simulink model "TestModel_V5_Timing_V2_2024a"  (R2024a)
settings: Solver=FixedStepAuto  StartTime=0.0  StopTime=40  FixedStep=1e-6  RelTol=1e-3
values from neighbouring files (symbols this model uses):
  par_Ctrl_FluxOffset = 0    [Param.m]
  par_Ctrl_MI = 0.99    [Param.m]
  par_Ctrl_SpdRt = 10    [Param.m]
  par_Ctrl_ThetaOffset = 0    [Param.m]
  par_IM_Frated = 50    [Param.m]
  par_IM_IratedPh = 7.9/sqrt(3)    [Param.m]
  par_IM_Lm = 0.527    [Param.m]
  par_IM_Lr = par_IM_Lm + par_IM_Llr    (= 0.5639)    [Param.m]
  par_IM_pp = 2    [Param.m]
  par_IM_Rs = 3.14    [Param.m]
  par_IM_VrmsLL = 400    [Param.m]
  par_uc_Ts = 100e-6    (= 0.0001)    [Param.m]
  pmsm = mcb.getPMSMParameters('Teknic2310P')    [mcb_pmsm_foc_sensorless_f28379d_datascript.m]
  Ts = T_pwm    (= 5e-05)    [mcb_pmsm_foc_sensorless_f28379d_datascript.m]
  Ts_motor = T_pwm/2    (= 2.5e-05)    [mcb_pmsm_foc_sensorless_f28379d_datascript.m]
undefined symbols (not defined in the file or in its folder): DiscIntNeverNeededParam, IM, par_pmsm_FluxLinkage, par_pmsm_Frated, par_pmsm_pp, par_pmsm_Vboost, par_pmsm_VrmsLL
libraries: spsOnDelayLib x24, mcbcontrolslib x12, spsTriangleGeneratorLib x4, autolibim x3, spsFirstOrderFilterLib x3, spsCurrentMeasurementLib x2, spsDCVoltageSourceLib x2, spsVoltageMeasurementLib x2, spsTwoLevelConverterLib x2, spsThreePhaseVIMeasurementLib x2, spsSeriesRLCBranchLib x1, sdolib x1
(part 1 of 3)
settings Model: PacingRate=1000  Creator=ckb527612  LastModifiedBy=ckb527612
settings ConfigComp: CovBoundaryAbsTol=1.0e-5

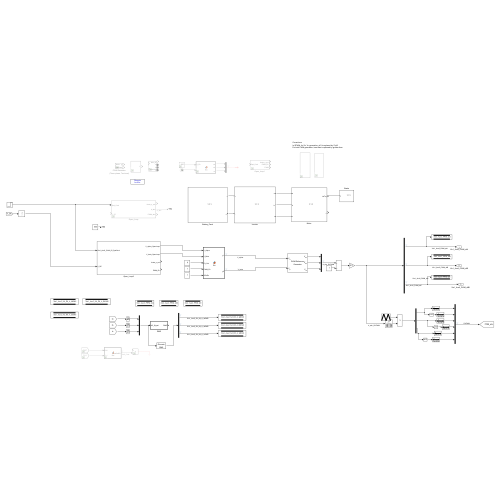
[thumbnail: Simulink's stored preview of the top-level diagram]
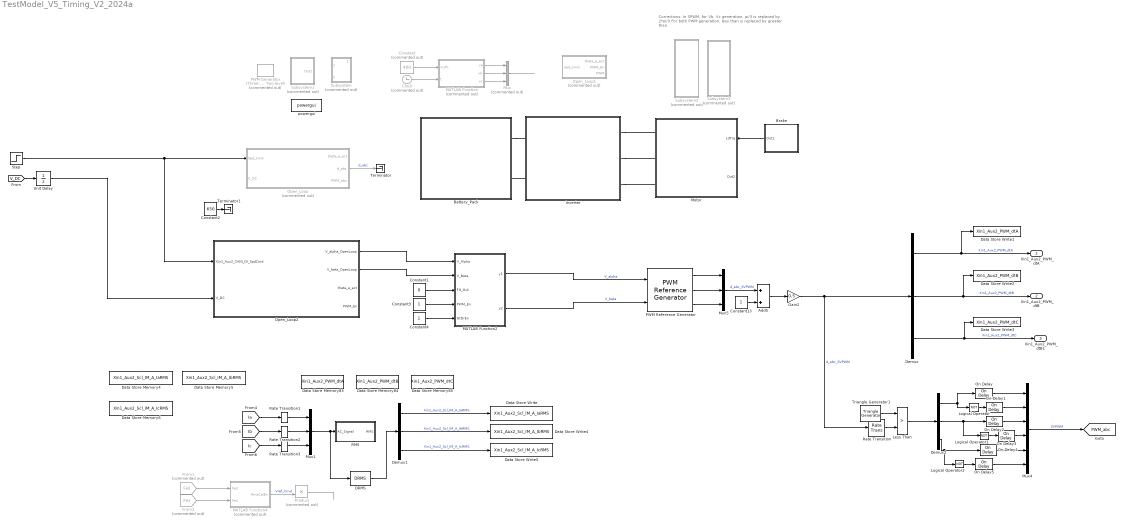
== system TestModel_V5_Timing_V2_2024a ==
  note: Corrections:
      | In SPWM, for Vb, Vc generation, pi/3 is replaced by 2*pi/3
      | For both PWM generation, less than is replaced by greater than
  Add5 : Sum
  Battery_Pack : Subsystem
      mask Display: image('battery_pack.jpg');
  Brake : Subsystem
      mask Display: image('brake-system-types-and-hydraulic-brake-parts-and-functions-6.png');
  Clock : Clock  Commented=on
  Constant : Constant  Commented=on  Value=400
  Constant1 : Constant  Value=0
  Constant13 : Constant
  Constant2 : Constant  Value=650
  Constant3 : Constant
  Constant4 : Constant
  DRMS : sdolib/RMS Blocks/DRMS  Ts=par_uc_Ts
  Data Store Memory4 : DataStoreMemory  DataStoreName=Xin1_Aux2_Scl_IM_A_IaRMS  WriteAfterWriteMsg=warning  ShowAdditionalParam=off
  Data Store Memory5 : DataStoreMemory  DataStoreName=Xin1_Aux2_Scl_IM_A_IbRMS  WriteAfterWriteMsg=warning  ShowAdditionalParam=off
  Data Store Memory6 : DataStoreMemory  DataStoreName=Xin1_Aux2_Scl_IM_A_IcRMS  WriteAfterWriteMsg=warning  ShowAdditionalParam=off
  Data Store Memory83 : DataStoreMemory  DataStoreName=Xin1_Aux2_PWM_dtA  WriteAfterWriteMsg=warning  ShowAdditionalParam=off
  Data Store Memory84 : DataStoreMemory  DataStoreName=Xin1_Aux2_PWM_dtB  WriteAfterWriteMsg=warning  ShowAdditionalParam=off
  Data Store Memory85 : DataStoreMemory  DataStoreName=Xin1_Aux2_PWM_dtC  WriteAfterWriteMsg=warning  ShowAdditionalParam=off
  Data Store Write : DataStoreWrite  DataStoreName=Xin1_Aux2_Scl_IM_A_IaRMS  IndexOptions=Index vector (dialog)  Indices=1  OutputSizes=1
  Data Store Write1 : DataStoreWrite  DataStoreName=Xin1_Aux2_PWM_dtA  IndexOptions=Index vector (dialog)  Indices=1  OutputSizes=1
  Data Store Write2 : DataStoreWrite  DataStoreName=Xin1_Aux2_PWM_dtB  IndexOptions=Index vector (dialog)  Indices=1  OutputSizes=1
  Data Store Write3 : DataStoreWrite  DataStoreName=Xin1_Aux2_PWM_dtC  IndexOptions=Index vector (dialog)  Indices=1  OutputSizes=1
  Data Store Write4 : DataStoreWrite  DataStoreName=Xin1_Aux2_Scl_IM_A_IbRMS  IndexOptions=Index vector (dialog)  Indices=1  OutputSizes=1
  Data Store Write5 : DataStoreWrite  DataStoreName=Xin1_Aux2_Scl_IM_A_IcRMS  IndexOptions=Index vector (dialog)  Indices=1  OutputSizes=1
  Demux : Demux  Outputs=3
  Demux1 : Demux  Outputs=3
  Demux2 : Demux  Outputs=3
  From1 : From  Commented=on  GotoTag=Fe2  TagVisibility=global
  From2 : From  Commented=on  GotoTag=Fe1  TagVisibility=global
  Gain2 : Gain  Gain=0.5
  Inverter : Subsystem
      mask Display: image('inverter.jpg');
  Less Than : RelationalOperator  Operator=>  OutDataTypeStr=boolean  RndMeth=Simplest  InputSameDT=off
  Logical Operator : Logic  Operator=NOT  AllPortsSameDT=off  OutDataTypeStr=boolean
  Logical Operator1 : Logic  Operator=NOT  AllPortsSameDT=off  OutDataTypeStr=boolean
  Logical Operator2 : Logic  Operator=NOT  AllPortsSameDT=off  OutDataTypeStr=boolean
  MATLAB Function : MATLAB Function  Commented=on  TreatAsAtomicUnit=on
  MATLAB Function2 : MATLAB Function  TreatAsAtomicUnit=on
  MATLAB Function4 : MATLAB Function  Commented=on  TreatAsAtomicUnit=on
  Motor : Subsystem
      settings: PortSchema="{\"entries\":[{\"content\":{\"sides\":[{\"content\":{\"connectorIds\":[\"LConn1\",\"LConn2\",\"LConn3\"]},\"type\":\"ConnectorPlacement.EquallySpacedRectSide\",\"uuid\":\"ba224176-031b-46fb-9c66-bda2665a14bd\"},{\"content\":{\"connectorIds\":[\"In1\",\"Out1\"],\"side\":\"RIGHT\"},\"type\":\"ConnectorPlacement.EquallySpacedRectSide\",\"uuid\":\"afd0beac-69db-400a-8bb3-39f53f6dd0dc\"},{\"content\":{\"side\":\"TOP\"},\"type\":\"ConnectorPlacement.EquallySpacedRectSide\",\"uuid\":\"9d949d83-5907-4238-9cb9-0d10379fcdec\"}]},\"type\":\"ConnectorPlacement.EquallySpacedConnector\",\"uuid\":\"43d01ac6-0c0f-4af8-b336-a00f131902fe\"}],\"packageUris\":[\"http://schema.mathworks.com/mf0/Connector/R2020b\"],\"version\":\"1.0\"}"
      mask Display: image('Motor3.jpg');
  Mux : Mux  Commented=on  Inputs=3
  Mux1 : Mux  Inputs=3
  Mux4 : Mux  Inputs=6
  Mux5 : Mux  Inputs=3
  On Delay{,1..5} (6 alike) : spsOnDelayLib/On Delay  DelayType=On delay  delay=3e-6  ic=0  Ts=1e-6
  Open_Loop : Subsystem  Commented=on
  Open_Loop1 : Subsystem  Commented=on
  Open_Loop2 : Subsystem
  "PWM Generator (Three-phase, Two-level)" : eePwmGeneratorTwoLevel/PWM Generator (Three-phase, Two-level)  Commented=on  PWMMode=Continuous PWM (CPWM)  CPWMMode=SVM: space vector modulation  DPWMMode=60 DPWM: 60 degree discontinuous PWM  fsw=10e3  Ts=1e-6
      settings: LibrarySourceBlock=|
      | ee_sl_lib/Pulse Width
      | Modulation/PWM Generator
      | (Three-phase, Two-level)
  PWM Reference Generator : mcbcontrolslib/PWM Reference Generator  inSignal=Valphabeta  modType=SVM: space vector modulation
      settings: LibrarySourceBlock=mcbhdllib/Controls/Math Transforms/PWM Reference Generator
  Product : Product  Commented=on
  RMS : Subsystem  TreatAsAtomicUnit=on
  Rate Transition : RateTransition
  Rate Transition1 : RateTransition  OutPortSampleTime=par_uc_Ts
  Rate Transition2 : RateTransition  OutPortSampleTime=par_uc_Ts
  Rate Transition3 : RateTransition  OutPortSampleTime=par_uc_Ts
  Step : Step  After=500
  Subsystem : Subsystem  Commented=on
  Subsystem1 : Subsystem  Commented=on
  Subsystem2 : Subsystem  Commented=on
  Subsystem3 : Subsystem  Commented=on
  Terminator : Terminator
  Terminator1 : Terminator
  Triangle Generator1 : spsTriangleGeneratorLib/Triangle Generator  Freq=10e3  Phase=0  Ts=1e-6
  Unit Delay : UnitDelay  SampleTime=-1  HasFrameUpgradeWarning=on
  powergui : spspowerguiLib/powergui  Priority=1  SimulationMode=Discrete  SampleTime=1e-6  frequency=60  Iterations=50  frequencyindice=0  Pbase=100e6  ErrMax=1e-4  UnitsV=kV  UnitsW=MW  buscounter=0  FunctionMessages=off  echomessages=off  EnableUseOfTLC=off  CurrentSourceSwitches=off  DisableSnubberDevices=off  DisableRonSwitches=off  DisableVfSwitches=off  DisplayEquations=off  AutomaticDiscreteSolvers=off  SolverType=Tustin/Backward Euler (TBE)  Interpol=off  ExternalGateDelay=off  methode=off  Ts=100  x0status=blocks  SPID=on  SwTol=0  HookPort=off  NonlinearTolerance=1e-4  nMaxIteration=100  ContinueOnMaxIteration=off  RestoreLinks=warning  ResistiveCurrentMeasurement=off  Frange=[0:2:500]  Ylog=off  Xlog=on  ShowGrid=off  save=off  variable=ZData  structure=0  ZoomFFT=off  StartTime=0.0  cycles=1  DisplayStyle=1  fundamental=60  FreqAxis=off  MaxFrequency=1000  frequencyindicesteady=1  RmsSteady=1  display=off
  Xin1_Aux2_PWM_dtA : Outport  VectorParamsAs1DForOutWhenUnconnected=off
  Xin1_Aux2_PWM_dtB : Outport  Port=2  VectorParamsAs1DForOutWhenUnconnected=off
  Xin1_Aux2_PWM_dtB1 : Outport  Port=3  VectorParamsAs1DForOutWhenUnconnected=off
  tag scope: PWM_abc=global
  wires:
  Constant/1 -> MATLAB Function/1(V_Ph)
  MATLAB Function/1(va) -> Mux/1
  MATLAB Function/2(vb) -> Mux/2
  MATLAB Function/3(vc) -> Mux/3
  Mux/1 -> ?
  Clock/1 -> MATLAB Function/2(t)
  Brake/1(Out1) -> Motor/1(LdTrq)
  Constant2/1 -> Terminator1/1
  Open_Loop/2(d_abc) -> Terminator/1  "d_abc"
  [V_DC] -> Unit Delay/1
  Unit Delay/1 -> Open_Loop2/2(V_DC)
  Step/1 -> Open_Loop2/1(Xin1_Aux2_CANI_DI_SpdCmd), Open_Loop/1(Spd_Cmd)
  MATLAB Function2/1(y1) -> PWM Reference Generator/1  "V_alpha"
  Constant3/1 -> MATLAB Function2/4(PWM_En)
  Constant13/1 -> Add5/2
  MATLAB Function2/2(y2) -> PWM Reference Generator/2  "V_beta"
  Demux/2 -> Data Store Write2/1, Xin1_Aux2_PWM_dtB/1  "Xin1_Aux2_PWM_dtB"
  Add5/1 -> Gain2/1
  Demux/3 -> Xin1_Aux2_PWM_dtB1/1, Data Store Write3/1  "Xin1_Aux2_PWM_dtC"
  Constant1/1 -> MATLAB Function2/3(Flt_Out)
  PWM Reference Generator/3 -> Mux5/3
  Open_Loop2/1(V_alpha_OpenLoop) -> MATLAB Function2/1(V_Alpha)
  Mux5/1 -> Add5/1  "d_abc_SVPWM"
  Open_Loop2/2(V_beta_OpenLoop) -> MATLAB Function2/2(V_Beta)
  PWM Reference Generator/2 -> Mux5/2
  Constant4/1 -> MATLAB Function2/5(GtDrEn)
  Demux/1 -> Data Store Write1/1, Xin1_Aux2_PWM_dtA/1  "Xin1_Aux2_PWM_dtA"
  PWM Reference Generator/1 -> Mux5/1
  [Ia] -> Rate Transition1/1
  [Ib] -> Rate Transition2/1
  Mux1/1 -> DRMS/1, RMS/1(AC_Signal)
  Demux1/1 -> Data Store Write/1  "Xin1_Aux2_Scl_IM_A_IaRMS"
  Demux1/3 -> Data Store Write5/1  "Xin1_Aux2_Scl_IM_A_IcRMS"
  [Ic] -> Rate Transition3/1
  DRMS/1 -> Demux1/1
  Demux1/2 -> Data Store Write4/1  "Xin1_Aux2_Scl_IM_A_IbRMS"
  Mux4/1 -> [PWM_abc]  "SVPWM"
  Logical Operator2/1 -> On Delay5/1
  On Delay5/1 -> Mux4/6
  Triangle Generator1/1 -> Less Than/1
  On Delay4/1 -> Mux4/5
  On Delay1/1 -> Mux4/2
  Logical Operator1/1 -> On Delay3/1
  Logical Operator/1 -> On Delay1/1
  Demux2/3 -> On Delay4/1, Logical Operator2/1
  Less Than/1 -> Demux2/1
  Demux2/1 -> Logical Operator/1, On Delay/1
  Demux2/2 -> On Delay2/1, Logical Operator1/1
  On Delay2/1 -> Mux4/3
  Gain2/1 -> Rate Transition/1, Demux/1  "d_abc_SVPWM"
  On Delay/1 -> Mux4/1
  On Delay3/1 -> Mux4/4
  Rate Transition/1 -> Less Than/2
  Rate Transition1/1 -> Mux1/1
  Rate Transition2/1 -> Mux1/2
  Rate Transition3/1 -> Mux1/3
  From1/1 -> MATLAB Function4/1(Fe2)
  From2/1 -> MATLAB Function4/2(Fe1)
  MATLAB Function4/1(RmsCalEn) -> Product/2  "Vref_Cmd"
  Product/1 -> ?
  connections:
  Inverter/LConn2 -- Battery_Pack/RConn2
  Inverter/RConn2 -- Motor/LConn2
  Inverter/RConn1 -- Motor/LConn1
  Battery_Pack/RConn1 -- Inverter/LConn1
  Inverter/RConn3 -- Motor/LConn3

== system TestModel_V5_Timing_V2_2024a/Battery_Pack ==
  Current Measurement : spsCurrentMeasurementLib/Current Measurement  PhasorSimulation=off  OutputType=Complex  PSBequivalent=0
  From : From  Commented=on  GotoTag=V_DC  TagVisibility=global
  Series RLC Branch : spsSeriesRLCBranchLib/Series RLC Branch  LConnTagsString=__new0  RConnTagsString=__new0  BranchType=RC  Resistance=0.4e-3  Inductance=1e-3  SetiL0=off  InitialCurrent=0  Capacitance=300e-6  Setx0=on  InitialVoltage=650  Measurements=None
  Terminator : Terminator
  "V_in " : spsDCVoltageSourceLib/DC Voltage Source  Amplitude=650  Measurements=None
  Voltage Measurement : spsVoltageMeasurementLib/Voltage Measurement  PhasorSimulation=off  OutputType=Complex  PSBequivalent=0
  - : PMIOPort  Side=Right
  -1 : PMIOPort  Port=2  Side=Right
  tag scope: I_in=global, V_DC=global
  wires:
  Current Measurement/1 -> [I_in]  "I_in"
  Voltage Measurement/1 -> [V_DC]  "V_DC"
  From/1 -> Terminator/1
  connections:
  Current Measurement/RConn1 -- -/RConn1
  Voltage Measurement/LConn1 -- Current Measurement/LConn1 -- "V_in "/RConn1 -- Series RLC Branch/LConn1
  -1/RConn1 -- Voltage Measurement/LConn2 -- "V_in "/LConn1 -- Series RLC Branch/RConn1

== system TestModel_V5_Timing_V2_2024a/Brake ==
  Constant : Constant  Commented=on  Value=pmsm.LdTrq
  Data Type Conversion : DataTypeConversion  Commented=on  OutDataTypeStr=single  SaturateOnIntegerOverflow=off  RndMeth=Floor
  IIR Filter : mcbcontrolslib/IIR Filter  VariantControl=Low Pass Filter  VariantSelect=Low-pass  FilterConstantInputType=Specify via dialog  Filter_constant=0.001  InitialOutput=Specify via dialog  InitialOutputValue=0  ExternalReset=none  advancedSettings=off  Ts=50e-6  cutOff_freq=3.1863
  T_load : Step  Before=IM.Tshaft*0  After=IM.Tshaft*0.15  SampleTime=1e-6
  T_load1 : Step  Commented=on  Time=2.5  Before=pmsm.T_rated*0.1  After=pmsm.T_rated*0.5  SampleTime=Ts_motor
  Terminator : Terminator
  Out1 : Outport
  wires:
  Constant/1 -> Terminator/1
  T_load/1 -> IIR Filter/1
  IIR Filter/1 -> Out1/1

== system TestModel_V5_Timing_V2_2024a/Inverter ==
  Constant2 : Constant  Value=0
  Data Type Conversion : DataTypeConversion  SaturateOnIntegerOverflow=off  RndMeth=Floor
  Two-Level Converter : spsTwoLevelConverterLib/Two-Level Converter  ModelType=Switching function  Ron=1e-3  Rs=1e6  Cs=inf  Vforward=[0,0]  Ron_Diode=1e-3  Rs_Diode=1e6  Cs_Diode=inf  Vf_Diode=0  Rs_CurrentSource=inf  Ron_ACsource=1e-3
  Universal Bridge : spsUniversalBridgeLib/Universal Bridge  Commented=on  Arms=3  SnubberResistance=1e5  SnubberCapacitance=inf  Device=IGBT / Diodes  Ron=1e-3  Lon=0  ForwardVoltages="[  0  0  ]"  ForwardVoltage=0  GTOparameters=[ 10e-6 , 20e-6 ]  IGBTparameters=[ 1e-6 , 2e-6 ]  Measurements=None  Measurements_2=None  converterType=Rectifier
  + : PMIOPort  Side=Left
  - : PMIOPort  Port=2  Side=Left
  a : PMIOPort  Port=3  Side=Right
  b : PMIOPort  Port=4  Side=Right
  c : PMIOPort  Port=5  Side=Right
  wires:
  Data Type Conversion/1 -> Two-Level Converter/1  "PWM"
  [PWM_abc] -> Data Type Conversion/1
  Constant2/1 -> Two-Level Converter/2
  connections:
  b/RConn1 -- Two-Level Converter/LConn2
  c/RConn1 -- Two-Level Converter/LConn3
  a/RConn1 -- Two-Level Converter/LConn1
  Two-Level Converter/RConn2 -- -/RConn1
  +/RConn1 -- Two-Level Converter/RConn1

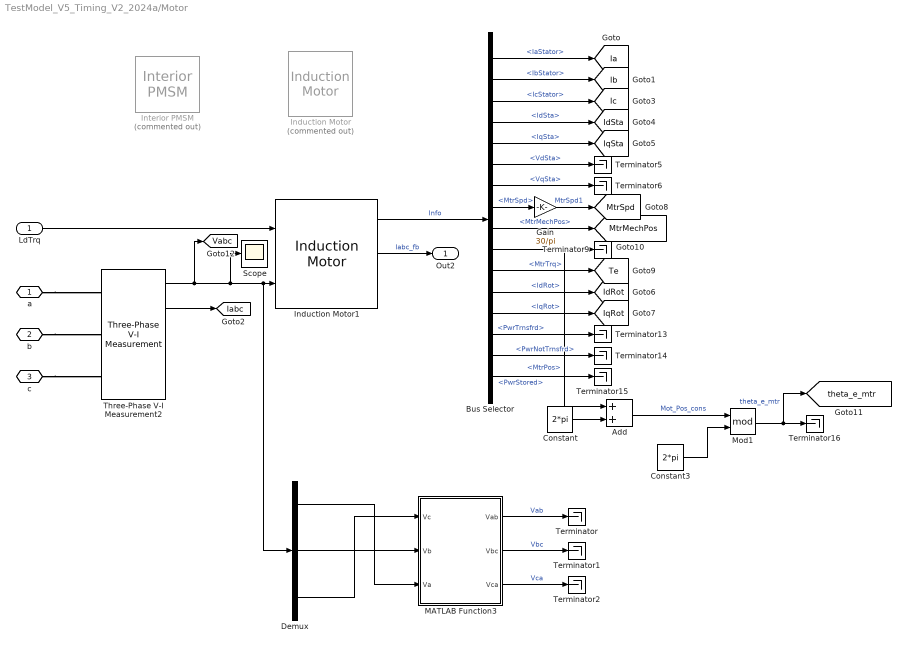
== system TestModel_V5_Timing_V2_2024a/Motor ==
  LdTrq : Inport
  Add : Sum
  Bus Selector : BusSelector  OutputSignals=IaStator,IbStator,IcStator,IdSta,IqSta,VdSta,VqSta,MtrSpd,MtrMechPos,MtrPos,MtrTrq,IdRot,IqRot,PwrInfo.PwrTrnsfrd,PwrInfo.PwrNotTrnsfrd,PwrInfo.PwrStored
  Constant : Constant  Value=2*pi
  Constant3 : Constant  Value=2*pi  OutDataTypeStr=double
  Demux : Demux  Outputs=3
  Gain : Gain  Gain=30/pi
  Induction Motor : autolibim/Induction Motor  Commented=on  sim_type=Discrete  Ts=0.001  port_config=Torque  P=2  Zs=[0.85 0.0139]  Zr="[0.55  0.0121]"  Lm=0.048  mechanical=[0.055 0.0078 0.5]  theta_init=0  omega_init=0  RefBlkName='autolibim/Induction Motor'  aMode=5
      settings: LibrarySourceBlock=mcblib/Electrical Systems/Motors/Induction Motor
  Induction Motor1 : autolibim/Induction Motor  sim_type=Discrete  Ts=1e-6  port_config=Torque  P=2  Zs=[3.14 0.0369]  Zr="[2.59  0.0369]"  Lm=0.527  mechanical=[0.01*10 0.00316 0.1]  theta_init=0  omega_init=0  RefBlkName='autolibim/Induction Motor'  aMode=5
      settings: LibrarySourceBlock=mcblib/Electrical Systems/Motors/Induction Motor
  Interior PMSM : autolibpmsminterior/Interior PMSM  Commented=on  port_config=Torque  sim_type=Continuous  Ts=0.001  FilePath=interiorpmsm_motordata.m  P=4  Rs=1.2  Ldq=[14.29e-3 23.15e-3]  KConstText=Permanent flux linkage constant (lambda_pm):  lambda_pm=0.5  Ke=159.9771  mechanical=[0.0045, 4.924e-4, 0]  idq0=[0 0]  theta_init=0  omega_init=0  KConst=0.1194  lambda_pm_calc=0.1194  Kt=1.323  RefBlkName='autolibpmsminterior/Interior PMSM'  aMode=1
      settings: LibrarySourceBlock=autolibemachines/Interior PMSM
  MATLAB Function3 : MATLAB Function  TreatAsAtomicUnit=on
  Mod1 : Math  Operator=mod
  Scope : Scope
  Terminator{,1..2,5..6,9,13..16} (10 alike) : Terminator
  Three-Phase V-I Measurement2 : spsThreePhaseVIMeasurementLib/Three-Phase V-I Measurement  VoltageMeasurement=phase-to-phase  SetLabelV=off  LabelV=Vabc  Vpu=off  VpuLL=off  CurrentMeasurement=yes  SetLabelI=off  LabelI=Iabc  Ipu=off  Pbase=100e6  Vbase=500e3  OutputType=Complex  PhasorSimulation=off  PSBequivalent=0
  a : PMIOPort  Side=Left
  b : PMIOPort  Port=2  Side=Left
  c : PMIOPort  Port=3  Side=Left
  Out2 : Outport
  tag scope: Ia=global, Iabc=global, Ib=global, Ic=global, IdRot=global, IdSta=global, IqRot=global, IqSta=global, MtrMechPos=global, MtrSpd=global, Te=global, Vabc=global, theta_e_mtr=global
  wires:
  Three-Phase V-I Measurement2/2 -> [Iabc]
  LdTrq/1 -> Induction Motor1/1
  Three-Phase V-I Measurement2/1 -> [Vabc], Scope/1, Demux/1, Induction Motor1/2
  Induction Motor1/1 -> Bus Selector/1  "Info"
  Bus Selector/1 -> [Ia]  "<IaStator>"
  Bus Selector/5 -> [IqSta]  "<IqSta>"
  Bus Selector/14 -> Terminator13/1  "<PwrTrnsfrd>"
  Bus Selector/6 -> Terminator5/1  "<VdSta>"
  Induction Motor1/2 -> Out2/1  "Iabc_fb"
  Gain/1 -> [MtrSpd]  "MtrSpd1"
  Bus Selector/12 -> [IdRot]  "<IdRot>"
  Bus Selector/10 -> Add/1, Terminator9/1  "<MtrPos>"
  Bus Selector/11 -> [Te]  "<MtrTrq>"
  Bus Selector/9 -> [MtrMechPos]  "<MtrMechPos>"
  Bus Selector/2 -> [Ib]  "<IbStator>"
  Bus Selector/4 -> [IdSta]  "<IdSta>"
  Bus Selector/13 -> [IqRot]  "<IqRot>"
  Bus Selector/15 -> Terminator14/1  "<PwrNotTrnsfrd>"
  Bus Selector/3 -> [Ic]  "<IcStator>"
  Bus Selector/16 -> Terminator15/1  "<PwrStored>"
  Bus Selector/7 -> Terminator6/1  "<VqSta>"
  Constant/1 -> Add/2
  Add/1 -> Mod1/1  "Mot_Pos_cons"
  Bus Selector/8 -> Gain/1  "<MtrSpd>"
  Demux/3 -> MATLAB Function3/1(Vc)
  MATLAB Function3/1(Vab) -> Terminator/1  "Vab"
  Demux/1 -> MATLAB Function3/3(Va)
  MATLAB Function3/3(Vca) -> Terminator2/1  "Vca"
  MATLAB Function3/2(Vbc) -> Terminator1/1  "Vbc"
  Demux/2 -> MATLAB Function3/2(Vb)
  Constant3/1 -> Mod1/2
  Mod1/1 -> [theta_e_mtr], Terminator16/1  "theta_e_mtr"
  connections:
  b/RConn1 -- Three-Phase V-I Measurement2/LConn2
  a/RConn1 -- Three-Phase V-I Measurement2/LConn1
  c/RConn1 -- Three-Phase V-I Measurement2/LConn3

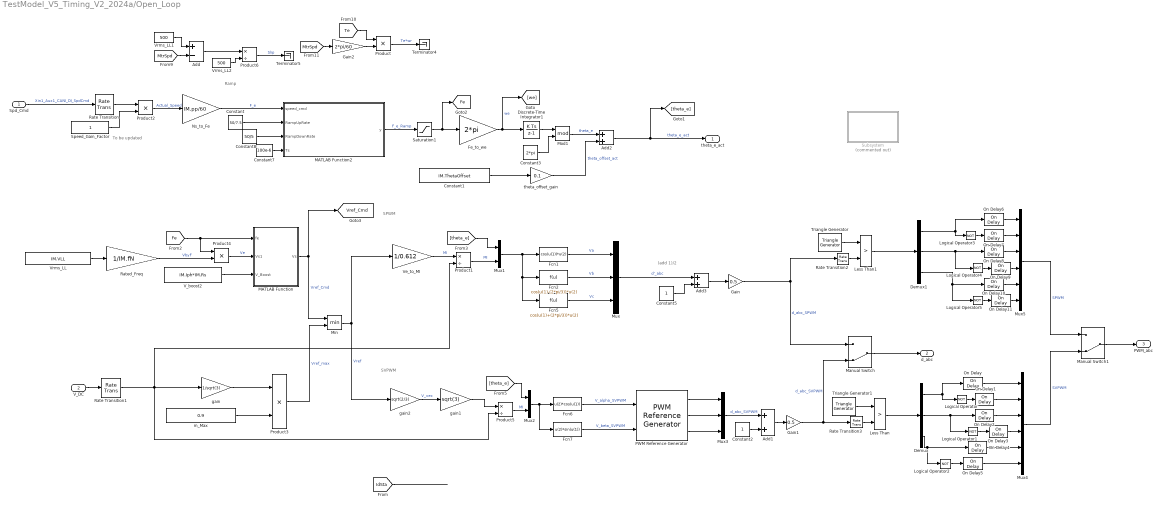
== system TestModel_V5_Timing_V2_2024a/Open_Loop ==
  note: Ramp
  note: SVPWM
  note: SPWM
  note: To be updated
  note: (add 1)/2
  Spd_Cmd : Inport
  V_DC : Inport  Port=2
  Add : Sum  Inputs=+-
  Add1 : Sum
  Add2 : Sum
  Add3 : Sum
  Constant : Constant  Value=50/7.5
  Constant1 : Constant  Value=IM.ThetaOffset
  Constant2 : Constant
  Constant3 : Constant  Value=2*pi  OutDataTypeStr=double
  Constant5 : Constant
  Constant7 : Constant  Value=100e-6
  Constant8 : Constant  Value=50/5
  Demux : Demux  Outputs=3
  Demux1 : Demux  Outputs=3
  Discrete-Time Integrator1 : DiscreteIntegrator  SampleTime=-1  OutDataTypeStr=double  ICPrevOutput=DiscIntNeverNeededParam  ICPrevScaledInput=DiscIntNeverNeededParam
  Fcn1 : Fcn  Expr=cos(u(1))*u(2)
  Fcn2 : Fcn  Expr=cos(u(1)-(2*pi/3))*u(2)
  Fcn5 : Fcn  Expr=cos(u(1)+(2*pi/3))*u(2)
  Fcn6 : Fcn  Expr=u(2)*cos(u(1))
  Fcn7 : Fcn  Expr=u(2)*sin(u(1))
  Fe_to_we : Gain  Gain=2*pi
  Gain : Gain  Gain=0.5
  Gain1 : Gain  Gain=0.5
  Gain2 : Gain  Gain=2*pi/60
  Less Than : RelationalOperator  Operator=>  OutDataTypeStr=boolean  RndMeth=Simplest  InputSameDT=off
  Less Than1 : RelationalOperator  Operator=>  OutDataTypeStr=boolean  RndMeth=Simplest  InputSameDT=off
  Logical Operator{,1..5} (6 alike) : Logic  Operator=NOT  AllPortsSameDT=off  OutDataTypeStr=boolean
  MATLAB Function : MATLAB Function  TreatAsAtomicUnit=on
  MATLAB Function2 : MATLAB Function  TreatAsAtomicUnit=on
  Manual Switch : ManualSwitch  CurrentSetting=0
  Manual Switch1 : ManualSwitch  CurrentSetting=0
  Min : MinMax  Inputs=2
  Mod1 : Math  Operator=mod
  Mux : Mux  Inputs=3
  Mux1 : Mux  Inputs=2
  Mux2 : Mux  Inputs=2
  Mux3 : Mux  Inputs=3
  Mux4 : Mux  Inputs=6
  Mux5 : Mux  Inputs=6
  Ns_to_Fe : Gain  Gain=IM.pp/60
  On Delay{,1..11} (12 alike) : spsOnDelayLib/On Delay  DelayType=On delay  delay=3e-6  ic=0  Ts=1e-6
  PWM Reference Generator : mcbcontrolslib/PWM Reference Generator  inSignal=Valphabeta  modType=SVM: space vector modulation
      settings: LibrarySourceBlock=mcbhdllib/Controls/Math Transforms/PWM Reference Generator
  Product{,2..4} (4 alike) : Product
  Product1 : Product  Inputs=*/
  Product5 : Product  Inputs=*/
  Product6 : Product  Inputs=*/
  Rate Transition : RateTransition  OutPortSampleTime=100e-6
  Rate Transition1 : RateTransition  OutPortSampleTime=100e-6
  Rate Transition2 : RateTransition  OutPortSampleTime=1e-6
  Rate Transition3 : RateTransition  OutPortSampleTime=1e-6
  Rated_Freq : Gain  Gain=1/IM.fN  ParamDataTypeStr=double  OutDataTypeStr=double
  Saturation1 : Saturate  UpperLimit=50  LowerLimit=0
  Speed_Gain_Factor : Constant
  Subsystem : Subsystem  Commented=on
  Terminator4 : Terminator
  Terminator5 : Terminator
  Triangle Generator : spsTriangleGeneratorLib/Triangle Generator  Freq=10e3  Phase=0  Ts=1e-6
  Triangle Generator1 : spsTriangleGeneratorLib/Triangle Generator  Freq=10e3  Phase=0  Ts=1e-6
  V_boost2 : Constant  Value=IM.Iph*IM.Rs
  Ve_to_MI : Gain  Gain=1/0.612  ParamDataTypeStr=double  OutDataTypeStr=double
  Vrms_LL : Constant  Value=IM.VLL  OutDataTypeStr=double
  Vrms_LL1 : Constant  Value=500  OutDataTypeStr=double
  Vrms_LL2 : Constant  Value=500  OutDataTypeStr=double
  gain : Gain  Gain=1/sqrt(3)
  gain1 : Gain  Gain=sqrt(3)
  gain2 : Gain  Gain=sqrt(2/3)
  m_Max : Constant  Value=0.9
  theta_offset_gain : Gain  Gain=0.1
  theta_e_act : Outport
  d_abc : Outport  Port=2
  PWM_abc : Outport  Port=3
  tag scope: Fe=global, Vref_Cmd=global
  wires:
  Product2/1 -> Ns_to_Fe/1  "Actual_Speed"
  Fe_to_we/1 -> Discrete-Time Integrator1/1, [we]  "we"
  Add2/1 -> theta_e_act/1, [theta_e]  "theta_e_act"
  Discrete-Time Integrator1/1 -> Mod1/1
  Mod1/1 -> Add2/1  "theta_e"
  Speed_Gain_Factor/1 -> Product2/2
  Ns_to_Fe/1 -> MATLAB Function2/1(speed_cmd)  "F_e"
  Constant3/1 -> Mod1/2
  theta_offset_gain/1 -> Add2/2  "theta_offset_act"
  Spd_Cmd/1 -> Rate Transition/1  "Xin1_Aux1_CANI_DI_SpdCmd"
  Constant1/1 -> theta_offset_gain/1
  Vrms_LL/1 -> Rated_Freq/1
  Rated_Freq/1 -> Product4/2  "VbyF"
  [Fe] -> Product4/1, MATLAB Function/1(fe)
  Product4/1 -> MATLAB Function/2(Vs1)  "Ve"
  Product1/1 -> Mux1/2  "MI"
  [theta_e] -> Mux1/1
  V_boost2/1 -> MATLAB Function/3(V_Boost)
  MATLAB Function/1(Vs) -> Min/1, [Vref_Cmd]  "Vref_Cmd"
  Ve_to_MI/1 -> Product1/1  "MI"
  Mux1/1 -> Fcn5/1, Fcn2/1, Fcn1/1
  Fcn1/1 -> Mux/1  "Va"
  Fcn2/1 -> Mux/2  "Vb"
  Fcn5/1 -> Mux/3  "Vc"
  Constant5/1 -> Add3/2
  Add3/1 -> Gain/1
  Mux/1 -> Add3/1  "d'_abc"
  Manual Switch/1 -> d_abc/1
  m_Max/1 -> Product3/2
  gain/1 -> Product3/1
  Product3/1 -> Min/2  "Vref_max"
  Min/1 -> gain2/1, Ve_to_MI/1  "Vref"
  gain1/1 -> Product5/1
  V_DC/1 -> Rate Transition1/1
  Product5/1 -> Mux2/2  "MI"
  [theta_e] -> Mux2/1
  Mux2/1 -> Fcn6/1, Fcn7/1
  Fcn6/1 -> PWM Reference Generator/1  "V_alpha_SVPWM"
  Fcn7/1 -> PWM Reference Generator/2  "V_beta_SVPWM"
  PWM Reference Generator/1 -> Mux3/1
  PWM Reference Generator/2 -> Mux3/2
  PWM Reference Generator/3 -> Mux3/3
  Gain1/1 -> Rate Transition3/1, Manual Switch/2  "d_abc_SVPWM"
  Gain/1 -> Rate Transition2/1, Manual Switch/1  "d_abc_SPWM"
  gain2/1 -> gain1/1  "V_vec"
  Add1/1 -> Gain1/1
  Constant2/1 -> Add1/2
  Mux3/1 -> Add1/1  "d_abc_SVPWM"
  Demux/1 -> Logical Operator/1, On Delay/1
  Logical Operator/1 -> On Delay1/1
  Logical Operator1/1 -> On Delay3/1
  Demux/2 -> On Delay2/1, Logical Operator1/1
  On Delay5/1 -> Mux4/6
  Demux/3 -> On Delay4/1, Logical Operator2/1
  Mux4/1 -> Manual Switch1/2  "SVPWM"
  Mux5/1 -> Manual Switch1/1  "SPWM"
  Demux1/3 -> On Delay10/1, Logical Operator5/1
  Demux1/2 -> On Delay8/1, Logical Operator4/1
  Demux1/1 -> On Delay6/1, Logical Operator3/1
  Logical Operator3/1 -> On Delay7/1
  Logical Operator4/1 -> On Delay9/1
  Logical Operator5/1 -> On Delay11/1
  Manual Switch1/1 -> PWM_abc/1
  Triangle Generator1/1 -> Less Than/1
  Less Than/1 -> Demux/1
  Triangle Generator/1 -> Less Than1/1
  Less Than1/1 -> Demux1/1
  On Delay/1 -> Mux4/1
  On Delay1/1 -> Mux4/2
  On Delay2/1 -> Mux4/3
  On Delay4/1 -> Mux4/5
  On Delay3/1 -> Mux4/4
  Logical Operator2/1 -> On Delay5/1
  Saturation1/1 -> Fe_to_we/1, [Fe]
  Constant/1 -> MATLAB Function2/2(RampUpRate)
  Constant8/1 -> MATLAB Function2/3(RampDownRate)
  Constant7/1 -> MATLAB Function2/4(Ts)
  MATLAB Function2/1(y) -> Saturation1/1  "F_e_Ramp"
  [IdSta] -> ?
  [MtrSpd] -> Add/2
  [MtrSpd] -> Gain2/1
  [Te] -> Product/1
  Product/1 -> Terminator4/1  "Te*wr"
  Vrms_LL1/1 -> Add/1
  Add/1 -> Product6/1
  Vrms_LL2/1 -> Product6/2
  Product6/1 -> Terminator5/1  "Slip"
  Gain2/1 -> Product/2
  On Delay6/1 -> Mux5/1
  On Delay7/1 -> Mux5/2
  On Delay8/1 -> Mux5/3
  On Delay9/1 -> Mux5/4
  On Delay10/1 -> Mux5/5
  On Delay11/1 -> Mux5/6
  Rate Transition1/1 -> gain/1, Product1/2, Product5/2
  Rate Transition/1 -> Product2/1
  Rate Transition2/1 -> Less Than1/2
  Rate Transition3/1 -> Less Than/2

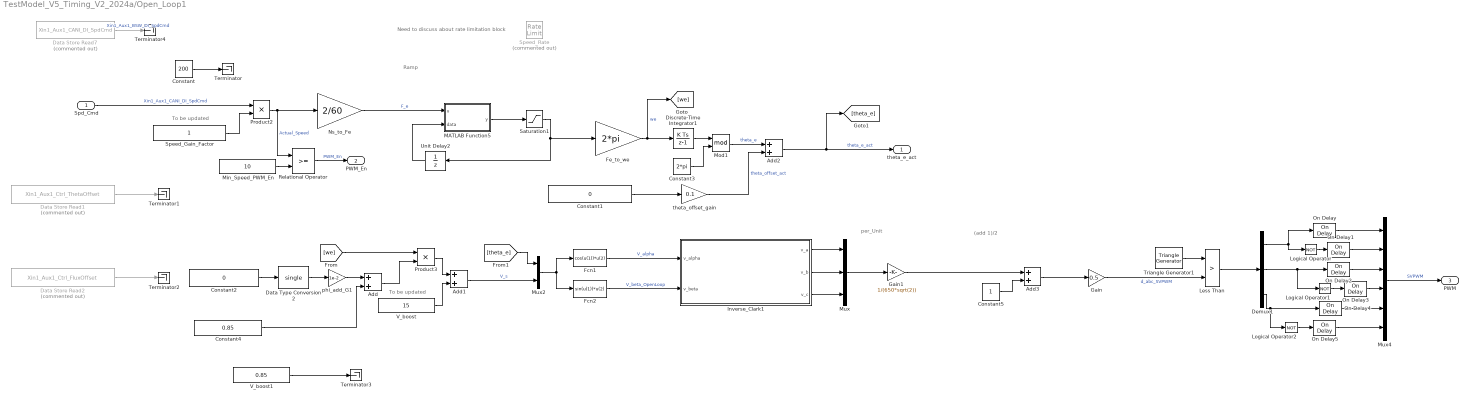
== system TestModel_V5_Timing_V2_2024a/Open_Loop1 ==
  note: Ramp
  note: Need to discuss about rate limitation block
  note: To be updated
  note: To be updated
  note: per_Unit
  note: (add 1)/2
  Spd_Cmd : Inport
  Add{,1..3} (4 alike) : Sum
  Constant : Constant  Value=200
  Constant1 : Constant  Value=0
  Constant2 : Constant  Value=0
  Constant3 : Constant  Value=2*pi  OutDataTypeStr=double
  Constant4 : Constant  Value=0.85  OutDataTypeStr=double
  Constant5 : Constant
  Data Store Read1 : DataStoreRead  Commented=on  DataStoreName=Xin1_Aux1_Ctrl_ThetaOffset  IndexOptions=Index vector (dialog)  Indices=1  OutputSizes=1
  Data Store Read2 : DataStoreRead  Commented=on  DataStoreName=Xin1_Aux1_Ctrl_FluxOffset  IndexOptions=Index vector (dialog)  Indices=1  OutputSizes=1
  Data Store Read7 : DataStoreRead  Commented=on  DataStoreName=Xin1_Aux1_CANI_DI_SpdCmd  IndexOptions=Index vector (dialog)  Indices=1  OutputSizes=1
  Data Type Conversion2 : DataTypeConversion  OutDataTypeStr=single  SaturateOnIntegerOverflow=off  RndMeth=Floor
  Demux1 : Demux  Outputs=3
  Discrete-Time Integrator1 : DiscreteIntegrator  SampleTime=-1  OutDataTypeStr=double  ICPrevOutput=DiscIntNeverNeededParam  ICPrevScaledInput=DiscIntNeverNeededParam
  Fcn1 : Fcn  Expr=cos(u(1))*u(2)
  Fcn2 : Fcn  Expr=sin(u(1))*u(2)
  Fe_to_we : Gain  Gain=2*pi
  Gain : Gain  Gain=0.5
  Gain1 : Gain  Gain=1/(650*sqrt(2))
  Inverse_Clark1 : MATLAB Function  TreatAsAtomicUnit=on
  Less Than : RelationalOperator  Operator=>  OutDataTypeStr=boolean  RndMeth=Simplest  InputSameDT=off
  Logical Operator : Logic  Operator=NOT  AllPortsSameDT=off  OutDataTypeStr=boolean
  Logical Operator1 : Logic  Operator=NOT  AllPortsSameDT=off  OutDataTypeStr=boolean
  Logical Operator2 : Logic  Operator=NOT  AllPortsSameDT=off  OutDataTypeStr=boolean
  MATLAB Function5 : MATLAB Function  TreatAsAtomicUnit=on
  Min_Speed_PWM_En : Constant  Value=10
  Mod1 : Math  Operator=mod
  Mux : Mux  Inputs=3
  Mux2 : Mux  Inputs=2
  Mux4 : Mux  Inputs=6
  Ns_to_Fe : Gain  Gain=2/60
  On Delay{,1..5} (6 alike) : spsOnDelayLib/On Delay  DelayType=On delay  delay=3e-6  ic=0  Ts=1e-6
  Product2 : Product
  Product3 : Product
  Relational Operator : RelationalOperator  OutDataTypeStr=boolean  RndMeth=Simplest  InputSameDT=off
  Saturation1 : Saturate  UpperLimit=100  LowerLimit=0
  Speed_Gain_Factor : Constant
  Speed_Rate : RateLimiter  Commented=on  RisingSlewLimit=par_Ctrl_SpdRt  FallingSlewLimit=-par_Ctrl_SpdRt  SampleTimeMode=inherited
  Terminator{,1..4} (5 alike) : Terminator
  Triangle Generator1 : spsTriangleGeneratorLib/Triangle Generator  Freq=10e3  Phase=0  Ts=1e-6
  Unit Delay2 : UnitDelay  SampleTime=-1  HasFrameUpgradeWarning=on
  V_boost : Constant  Value=15
  V_boost1 : Constant  Value=0.85
  phi_add_G1 : Gain  Gain=1e-2  ParamDataTypeStr=double  OutDataTypeStr=double
  theta_offset_gain : Gain  Gain=0.1
  theta_e_act : Outport
  PWM_En : Outport  Port=2
  PWM : Outport  Port=3
  wires:
  Product2/1 -> Relational Operator/1, Ns_to_Fe/1  "Actual_Speed"
  Mux2/1 -> Fcn2/1, Fcn1/1
  Fe_to_we/1 -> Discrete-Time Integrator1/1, [we]  "we"
  Constant4/1 -> Add/2
  Add/1 -> Product3/2
  Add2/1 -> theta_e_act/1, [theta_e]  "theta_e_act"
  Discrete-Time Integrator1/1 -> Mod1/1
  Product3/1 -> Add1/1
  [theta_e] -> Mux2/1
  [we] -> Product3/1
  Fcn2/1 -> Inverse_Clark1/2(v_beta)  "V_beta_OpenLoop"
  Mod1/1 -> Add2/1  "theta_e"
  Data Type Conversion2/1 -> phi_add_G1/1
  Speed_Gain_Factor/1 -> Product2/2
  V_boost/1 -> Add1/2
  Ns_to_Fe/1 -> MATLAB Function5/1(u)  "F_e"
  Constant3/1 -> Mod1/2
  theta_offset_gain/1 -> Add2/2  "theta_offset_act"
  phi_add_G1/1 -> Add/1
  Add1/1 -> Mux2/2  "V_s"
  Data Store Read2/1 -> Terminator2/1
  Data Store Read1/1 -> Terminator1/1
  Spd_Cmd/1 -> Product2/1  "Xin1_Aux1_CANI_DI_SpdCmd"
  MATLAB Function5/1(y) -> Saturation1/1
  Unit Delay2/1 -> MATLAB Function5/2(data)
  Saturation1/1 -> Unit Delay2/1, Fe_to_we/1
  Constant1/1 -> theta_offset_gain/1
  Constant2/1 -> Data Type Conversion2/1
  V_boost1/1 -> Terminator3/1
  Constant/1 -> Terminator/1
  Min_Speed_PWM_En/1 -> Relational Operator/2
  Relational Operator/1 -> PWM_En/1  "PWM_En"
  Data Store Read7/1 -> Terminator4/1  "Xin1_Aux1_BSW_DI_SpdCmd"
  Fcn1/1 -> Inverse_Clark1/1(v_alpha)  "V_alpha"
  Inverse_Clark1/2(v_b) -> Mux/2
  Constant5/1 -> Add3/2
  Inverse_Clark1/1(v_a) -> Mux/1
  Mux/1 -> Gain1/1
  Gain1/1 -> Add3/1
  Inverse_Clark1/3(v_c) -> Mux/3
  Add3/1 -> Gain/1
  Mux4/1 -> PWM/1  "SVPWM"
  Triangle Generator1/1 -> Less Than/1
  On Delay/1 -> Mux4/1
  Logical Operator/1 -> On Delay1/1
  Demux1/3 -> On Delay4/1, Logical Operator2/1
  Logical Operator2/1 -> On Delay5/1
  On Delay2/1 -> Mux4/3
  On Delay5/1 -> Mux4/6
  On Delay1/1 -> Mux4/2
  Logical Operator1/1 -> On Delay3/1
  Gain/1 -> Less Than/2  "d_abc_SVPWM"
  On Delay3/1 -> Mux4/4
  Demux1/2 -> On Delay2/1, Logical Operator1/1
  On Delay4/1 -> Mux4/5
  Demux1/1 -> Logical Operator/1, On Delay/1
  Less Than/1 -> Demux1/1

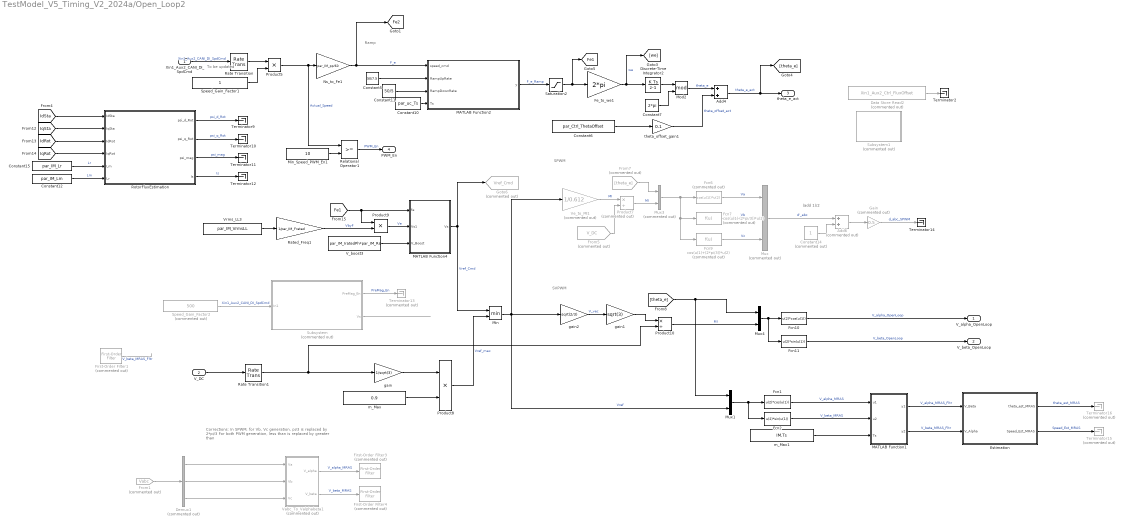
== system TestModel_V5_Timing_V2_2024a/Open_Loop2 ==
  note: To be updated
  note: Ramp
  note: SPWM
  note: Corrections:
      | In SPWM, for Vb, Vc generation, pi/3 is replaced by 2*pi/3
      | For both PWM generation, less than is replaced by greater than
  note: SVPWM
  note: (add 1)/2
  Xin1_Aux2_CANI_DI_SpdCmd : Inport
  V_DC : Inport  Port=2
  Add4 : Sum
  Add6 : Sum  Commented=on
  Constant10 : Constant  Value=par_uc_Ts
  Constant11 : Constant  Value=50/5  SampleTime=par_uc_Ts
  Constant12 : Constant  Value=par_IM_Lm  SampleTime=-1
  Constant14 : Constant  Commented=on
  Constant15 : Constant  Value=par_IM_Lr  SampleTime=-1
  Constant5 : Constant  Value=50/7.5  SampleTime=par_uc_Ts
  Constant6 : Constant  Value=par_Ctrl_ThetaOffset
  Constant7 : Constant  Value=2*pi  OutDataTypeStr=double
  Data Store Read2 : DataStoreRead  Commented=on  DataStoreName=Xin1_Aux2_Ctrl_FluxOffset  IndexOptions=Index vector (dialog)  Indices=1  OutputSizes=1
  Demux1 : Demux  Commented=on  Outputs=3
  Discrete-Time Integrator2 : DiscreteIntegrator  SampleTime=-1  OutDataTypeStr=double  ICPrevOutput=DiscIntNeverNeededParam  ICPrevScaledInput=DiscIntNeverNeededParam
  Estimation : Subsystem
  Fcn1 : Fcn  Expr=u(2)*cos(u(1))
  Fcn10 : Fcn  Expr=u(2)*cos(u(1))
  Fcn11 : Fcn  Expr=u(2)*sin(u(1))
  Fcn2 : Fcn  Expr=u(2)*sin(u(1))
  Fcn6 : Fcn  Commented=on  Expr=cos(u(1))*u(2)
  Fcn7 : Fcn  Commented=on  Expr=cos(u(1)-(2*pi/3))*u(2)
  Fcn9 : Fcn  Commented=on  Expr=cos(u(1)+(2*pi/3))*u(2)
  Fe_to_we1 : Gain  Gain=2*pi
  First-Order Filter1 : spsFirstOrderFilterLib/First-Order Filter  Commented=on  FilterType=Lowpass  Tc=1/80  Ts=IM.Ts  Initialize=off  Vac_Init=[0, 0, 60]  Vdc_Init=0  PlotResponse=off  FreqRange="[0,  200,  1]"
  First-Order Filter3 : spsFirstOrderFilterLib/First-Order Filter  Commented=on  FilterType=Lowpass  Tc=1/80  Ts=IM.Ts  Initialize=off  Vac_Init=[0, 0, 60]  Vdc_Init=0  PlotResponse=off  FreqRange="[0,  200,  1]"
  First-Order Filter4 : spsFirstOrderFilterLib/First-Order Filter  Commented=on  FilterType=Lowpass  Tc=1/80  Ts=IM.Ts  Initialize=off  Vac_Init=[0, 0, 60]  Vdc_Init=0  PlotResponse=off  FreqRange="[0,  200,  1]"
  From1 : From  Commented=on  GotoTag=Vabc  TagVisibility=global
  From5 : From  Commented=on  GotoTag=V_DC  TagVisibility=global
  From7 : From  Commented=on  GotoTag=theta_e
  Gain : Gain  Commented=on  Gain=0.5
  Goto6 : Goto  Commented=on  GotoTag=Vref_Cmd  TagVisibility=global
  MATLAB Function1 : MATLAB Function  TreatAsAtomicUnit=on
  MATLAB Function2 : MATLAB Function  TreatAsAtomicUnit=on
  MATLAB Function4 : MATLAB Function  TreatAsAtomicUnit=on
  Min : MinMax  Inputs=2
  Min_Speed_PWM_En1 : Constant  Value=10  SampleTime=par_uc_Ts
  Mod2 : Math  Operator=mod
  Mux : Mux  Commented=on  Inputs=3
  Mux1 : Mux  Inputs=2
  Mux3 : Mux  Commented=on  Inputs=2
  Mux4 : Mux  Inputs=2
  Ns_to_Fe1 : Gain  Gain=par_IM_pp/60
  Product10 : Product  Inputs=*/
  Product5 : Product
  Product7 : Product  Commented=on  Inputs=*/
  Product8 : Product
  Product9 : Product
  Rate Transition : RateTransition  OutPortSampleTime=par_uc_Ts
  Rate Transition1 : RateTransition  OutPortSampleTime=par_uc_Ts
  Rated_Freq1 : Gain  Gain=1/par_IM_Frated  ParamDataTypeStr=double  OutDataTypeStr=double
  Relational Operator1 : RelationalOperator  OutDataTypeStr=boolean  RndMeth=Simplest  InputSameDT=off
  RotorFluxEstimation : MATLAB Function  TreatAsAtomicUnit=on
  Saturation2 : Saturate  UpperLimit=50  LowerLimit=0
  Speed_Gain_Factor1 : Constant  SampleTime=par_uc_Ts
  Speed_Gain_Factor2 : Constant  Commented=on  Value=500
  Subsystem : Subsystem  Commented=on
  Subsystem1 : Subsystem  Commented=on
  Terminator{2,9..12,14} (6 alike) : Terminator
  Terminator13 : Terminator  Commented=on
  Terminator15 : Terminator  Commented=on
  Terminator16 : Terminator  Commented=on
  V_boost3 : Constant  Value=par_IM_IratedPh*par_IM_Rs  SampleTime=par_uc_Ts
  Vabc_To_Valphabeta1 : Subsystem  Commented=on
  Ve_to_MI1 : Gain  Commented=on  Gain=1/0.612  ParamDataTypeStr=double  OutDataTypeStr=double
  Vrms_LL3 : Constant  Value=par_IM_VrmsLL  OutDataTypeStr=double  SampleTime=par_uc_Ts
  gain : Gain  Gain=1/sqrt(3)
  gain1 : Gain  Gain=sqrt(3)
  gain2 : Gain  Gain=sqrt(2/3)
  m_Max : Constant  Value=0.9  SampleTime=par_uc_Ts
  m_Max1 : Constant  Value=IM.Ts  SampleTime=par_uc_Ts
  theta_offset_gain1 : Gain  Gain=0.1
  V_alpha_OpenLoop : Outport
  V_beta_OpenLoop : Outport  Port=2
  theta_e_act : Outport  Port=3
  PWM_En : Outport  Port=4
  tag scope: Fe1=global, Fe2=global
  wires:
  Data Store Read2/1 -> Terminator2/1
  Fcn10/1 -> V_alpha_OpenLoop/1  "V_alpha_OpenLoop"
  Fcn11/1 -> V_beta_OpenLoop/1  "V_beta_OpenLoop"
  Add4/1 -> theta_e_act/1, [theta_e]  "theta_e_act"
  Constant10/1 -> MATLAB Function2/4(Ts)
  Xin1_Aux2_CANI_DI_SpdCmd/1 -> Rate Transition/1  "Xin1_Aux2_CANI_DI_SpdCmd"
  theta_offset_gain1/1 -> Add4/2  "theta_offset_act"
  Saturation2/1 -> Fe_to_we1/1, [Fe1]
  Discrete-Time Integrator2/1 -> Mod2/1
  Mod2/1 -> Add4/1  "theta_e"
  Fe_to_we1/1 -> Discrete-Time Integrator2/1, [we]  "we"
  Speed_Gain_Factor1/1 -> Product5/2
  MATLAB Function2/1(y) -> Saturation2/1  "F_e_Ramp"
  Constant6/1 -> theta_offset_gain1/1
  Constant7/1 -> Mod2/2
  Ns_to_Fe1/1 -> [Fe2], MATLAB Function2/1(speed_cmd)  "F_e"
  Constant5/1 -> MATLAB Function2/2(RampUpRate)
  Constant11/1 -> MATLAB Function2/3(RampDownRate)
  Subsystem/2(Vs) -> ?
  Subsystem/1(PreMag_En) -> Terminator13/1  "PreMag_En"
  [IqSta] -> RotorFluxEstimation/2(IqSta)
  RotorFluxEstimation/2(psi_q_Rot) -> Terminator10/1  "psi_q_Rot"
  Gain/1 -> Terminator14/1  "d_abc_SPWM"
  Estimation/1(theta_est_MRAS) -> Terminator16/1  "theta_est_MRAS"
  Vrms_LL3/1 -> Rated_Freq1/1
  [theta_e] -> Mux1/1, Mux4/1
  Product7/1 -> Mux3/2  "MI"
  RotorFluxEstimation/1(psi_d_Rot) -> Terminator9/1  "psi_d_Rot"
  RotorFluxEstimation/4(Is) -> Terminator12/1  "Is"
  Fcn9/1 -> Mux/3  "Vc"
  gain/1 -> Product8/1
  V_DC/1 -> Rate Transition1/1
  Product9/1 -> MATLAB Function4/2(Vs1)  "Ve"
  Speed_Gain_Factor2/1 -> Subsystem/1(In1)  "Xin1_Aux2_CANI_DI_SpdCmd"
  Ve_to_MI1/1 -> Product7/1  "MI"
  V_boost3/1 -> MATLAB Function4/3(V_Boost)
  Constant12/1 -> RotorFluxEstimation/6(Lr)  "Lm"
  Product8/1 -> Min/2  "Vref_max"
  [IqRot] -> RotorFluxEstimation/4(IqRot)
  [IdSta] -> RotorFluxEstimation/1(IdSta)
  From5/1 -> Product7/2
  Product10/1 -> Mux4/2  "MI"
  MATLAB Function4/1(Vs) -> Goto6/1, Min/1  "Vref_Cmd"
  m_Max/1 -> Product8/2
  [IdRot] -> RotorFluxEstimation/3(IdRot)
  Mux3/1 -> Fcn9/1, Fcn7/1, Fcn6/1
  Constant14/1 -> Add6/2
  Min/1 -> Mux1/2, Ve_to_MI1/1, gain2/1  "Vref"
  Rated_Freq1/1 -> Product9/2  "VbyF"
  Mux/1 -> Add6/1  "d'_abc"
  gain2/1 -> gain1/1  "V_vec"
  Add6/1 -> Gain/1
  gain1/1 -> Product10/1
  Constant15/1 -> RotorFluxEstimation/5(Lm)  "Lr"
  RotorFluxEstimation/3(psi_mag) -> Terminator11/1  "psi_mag"
  From7/1 -> Mux3/1
  Fcn6/1 -> Mux/1  "Va"
  Fcn7/1 -> Mux/2  "Vb"
  Estimation/2(Speed_Est_MRAS) -> Terminator15/1  "Speed_Est_MRAS"
  [Fe1] -> Product9/1, MATLAB Function4/1(fe)
  Mux4/1 -> Fcn10/1, Fcn11/1
  Relational Operator1/1 -> PWM_En/1  "PWM_En"
  Min_Speed_PWM_En1/1 -> Relational Operator1/2
  Product5/1 -> Relational Operator1/1, Ns_to_Fe1/1  "Actual_Speed"
  Rate Transition/1 -> Product5/1
  Rate Transition1/1 -> Product10/2, gain/1
  MATLAB Function1/1(y1) -> Estimation/1(V_Beta)  "V_alpha_MRAS_Fltr"
  MATLAB Function1/2(y2) -> Estimation/2(V_Alpha)  "V_beta_MRAS_Fltr"
  First-Order Filter1/1 -> ?  "V_beta_MRAS_Fltr"
  From1/1 -> Demux1/1
  Demux1/3 -> Vabc_To_Valphabeta1/3(Vc)
  Demux1/2 -> Vabc_To_Valphabeta1/2(Vb)
  Vabc_To_Valphabeta1/2(V_beta) -> First-Order Filter4/1  "V_beta_MRAS"
  Vabc_To_Valphabeta1/1(V_alpha) -> First-Order Filter3/1  "V_alpha_MRAS"
  Demux1/1 -> Vabc_To_Valphabeta1/1(Va)
  Mux1/1 -> Fcn2/1, Fcn1/1
  Fcn1/1 -> MATLAB Function1/1(u1)  "V_alpha_MRAS"
  Fcn2/1 -> MATLAB Function1/2(u2)  "V_beta_MRAS"
  m_Max1/1 -> MATLAB Function1/3(Ts)

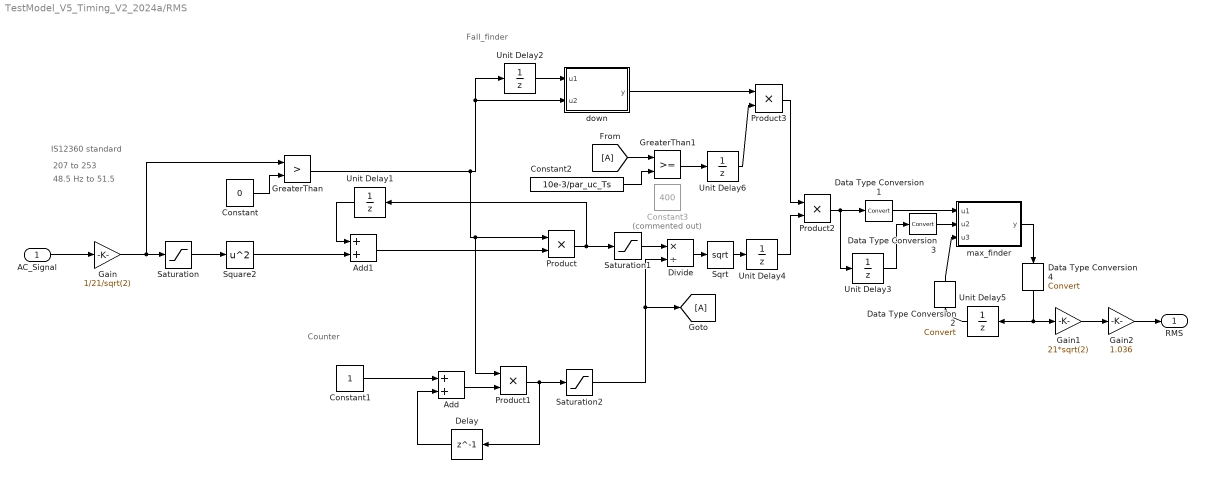
== system TestModel_V5_Timing_V2_2024a/RMS ==
  note: 207 to 253
  note: 48.5 Hz to 51.5
  note: IS12360 standard
  note: Counter
  note: Fall_finder
  AC_Signal : Inport
  Add : Sum
  Add1 : Sum
  Constant : Constant  Value=0
  Constant1 : Constant
  Constant2 : Constant  Value=10e-3/par_uc_Ts
  Constant3 : Constant  Commented=on  Value=400
  Data Type Conversion{1..4} (4 alike) : DataTypeConversion  SaturateOnIntegerOverflow=off  RndMeth=Floor
  Delay : Delay  DelayLength=1
  Divide : Product  Inputs=*/
  From : From
  Gain : Gain  Gain=1/21/sqrt(2)
  Gain1 : Gain  Gain=21*sqrt(2)
  Gain2 : Gain  Gain=1.036
  Goto : Goto
  GreaterThan : RelationalOperator  Operator=>  OutDataTypeStr=boolean  RndMeth=Simplest  InputSameDT=off
  GreaterThan1 : RelationalOperator  OutDataTypeStr=boolean  RndMeth=Simplest  InputSameDT=off
  Product{,1..3} (4 alike) : Product
  Saturation : Saturate  UpperLimit=6  LowerLimit=0.01
  Saturation1 : Saturate  UpperLimit=50000  LowerLimit=1
  Saturation2 : Saturate  UpperLimit=5000  LowerLimit=0.1
  Sqrt : Sqrt
  Square2 : Math  Operator=square
  Unit Delay{1..6} (6 alike) : UnitDelay  SampleTime=-1  HasFrameUpgradeWarning=on
  down : MATLAB Function  TreatAsAtomicUnit=on
  max_finder : MATLAB Function  TreatAsAtomicUnit=on
  RMS : Outport
  wires:
  Data Type Conversion4/1 -> Gain1/1, Unit Delay5/1
  Data Type Conversion3/1 -> max_finder/2(u2)
  Data Type Conversion1/1 -> max_finder/1(u1)
  Data Type Conversion2/1 -> max_finder/3(u3)
  max_finder/1(y) -> Data Type Conversion4/1
  Unit Delay6/1 -> Product3/2
  Product3/1 -> Product2/1
  GreaterThan1/1 -> Unit Delay6/1
  Constant2/1 -> GreaterThan1/2
  From/1 -> GreaterThan1/1
  down/1(y) -> Product3/1
  Gain1/1 -> Gain2/1
  AC_Signal/1 -> Gain/1
  Unit Delay2/1 -> down/1(u1)
  Sqrt/1 -> Unit Delay4/1
  Saturation2/1 -> Divide/2, Goto/1
  Product1/1 -> Delay/1, Saturation2/1
  Saturation1/1 -> Divide/1
  Unit Delay3/1 -> Data Type Conversion3/1
  Saturation/1 -> Square2/1
  Divide/1 -> Sqrt/1
  Constant/1 -> GreaterThan/2
  Constant1/1 -> Add/1
  Product/1 -> Saturation1/1, Unit Delay1/1
  Gain/1 -> GreaterThan/1, Saturation/1
  GreaterThan/1 -> Unit Delay2/1, down/2(u2), Product/1, Product1/1
  Unit Delay4/1 -> Product2/2
  Product2/1 -> Data Type Conversion1/1, Unit Delay3/1
  Delay/1 -> Add/2
  Unit Delay5/1 -> Data Type Conversion2/1
  Unit Delay1/1 -> Add1/1
  Add1/1 -> Product/2
  Add/1 -> Product1/2
  Square2/1 -> Add1/2
  Gain2/1 -> RMS/1

== system TestModel_V5_Timing_V2_2024a/Subsystem ==
  "  " : Inport
  PhaseVolt : Inport  Port=2
  Brake : Subsystem
      mask Display: image('brake-system-types-and-hydraulic-brake-parts-and-functions-6.png');
  Bus Selector : BusSelector  OutputSignals=MtrPos,IaStator,IbStator,IcStator,MtrSpd
  Constant2 : Constant  Value=0
  Current Measurement : spsCurrentMeasurementLib/Current Measurement  PhasorSimulation=off  OutputType=Complex  PSBequivalent=0
  Induction Motor : autolibim/Induction Motor  sim_type=Discrete  Ts=0.001  port_config=Torque  P=2  Zs=[0.85 0.0139]  Zr="[0.55  0.0121]"  Lm=0.048  mechanical=[0.055 0.0078 0.5]  theta_init=0  omega_init=0  RefBlkName='autolibim/Induction Motor'  aMode=5
      settings: LibrarySourceBlock=mcblib/Electrical Systems/Motors/Induction Motor
  Terminator{1..7} (7 alike) : Terminator
  Three-Phase V-I Measurement2 : spsThreePhaseVIMeasurementLib/Three-Phase V-I Measurement  VoltageMeasurement=phase-to-phase  SetLabelV=off  LabelV=Vabc  Vpu=off  VpuLL=off  CurrentMeasurement=yes  SetLabelI=off  LabelI=Iabc  Ipu=off  Pbase=100e6  Vbase=500e3  OutputType=Complex  PhasorSimulation=off  PSBequivalent=0
  Two-Level Converter : spsTwoLevelConverterLib/Two-Level Converter  ModelType=Switching devices  Ron=1e-3  Rs=1e6  Cs=inf  Vforward=[0,0]  Ron_Diode=1e-3  Rs_Diode=1e6  Cs_Diode=inf  Vf_Diode=1e-3  Rs_CurrentSource=inf  Ron_ACsource=1e-3
      settings: LibrarySourceBlock=sps_lib/Power Electronics/Two-Level Converter
  "V_in " : spsDCVoltageSourceLib/DC Voltage Source  Amplitude=650  Measurements=None
  Voltage Measurement : spsVoltageMeasurementLib/Voltage Measurement  PhasorSimulation=off  OutputType=Complex  PSBequivalent=0
  a : PMIOPort  Side=Right
  b : PMIOPort  Port=2  Side=Right
  c : PMIOPort  Port=3  Side=Right
  Iabc_fb : Outport
  tag scope: I_in=global, Iabc=global, V_in=global
  wires:
  Bus Selector/2 -> Terminator3/1  "<IaStator>"
  Voltage Measurement/1 -> [V_in]
  Bus Selector/1 -> Terminator2/1  "<MtrPos>"
  Three-Phase V-I Measurement2/2 -> [Iabc]
  Brake/1(Out1) -> Induction Motor/1
  Induction Motor/2 -> Iabc_fb/1  "Iabc_fb"
  Bus Selector/5 -> Terminator6/1  "<MtrSpd>"
  Current Measurement/1 -> [I_in]
  Bus Selector/3 -> Terminator4/1  "<IbStator>"
  "  "/1 -> Two-Level Converter/1
  Induction Motor/1 -> Bus Selector/1
  Three-Phase V-I Measurement2/1 -> Terminator7/1
  Bus Selector/4 -> Terminator5/1  "<IcStator>"
  Constant2/1 -> Two-Level Converter/2
  Induction Motor/3 -> Terminator1/1
  PhaseVolt/1 -> Induction Motor/2
  connections:
  Two-Level Converter/LConn2 -- Three-Phase V-I Measurement2/LConn2
  Voltage Measurement/LConn2 -- "V_in "/LConn1 -- Two-Level Converter/RConn2
  Two-Level Converter/LConn1 -- Three-Phase V-I Measurement2/LConn1
  Three-Phase V-I Measurement2/RConn3 -- c/RConn1
  Two-Level Converter/LConn3 -- Three-Phase V-I Measurement2/LConn3
  "V_in "/RConn1 -- Voltage Measurement/LConn1 -- Current Measurement/LConn1
  Current Measurement/RConn1 -- Two-Level Converter/RConn1
  Three-Phase V-I Measurement2/RConn2 -- b/RConn1
  Three-Phase V-I Measurement2/RConn1 -- a/RConn1

== system TestModel_V5_Timing_V2_2024a/Subsystem1 ==
  Add1 : Sum
  Constant : Constant  Value=1000
  Constant1 : Constant  Value=-pi/20*10
  Data Type Conversion1 : DataTypeConversion  SaturateOnIntegerOverflow=off  RndMeth=Floor
  Data Type Conversion2 : DataTypeConversion  SaturateOnIntegerOverflow=off  RndMeth=Floor
  Data Type Conversion3 : DataTypeConversion  SaturateOnIntegerOverflow=off  RndMeth=Floor
  Gain2 : Gain  Gain=2*2/120*2*pi
  Gain3 : Gain  Gain=pmsm.Ke*sqrt(3)/1000/450
  Logical Operator : Logic  Operator=NOT  AllPortsSameDT=off  OutDataTypeStr=boolean
  Logical Operator1 : Logic  Operator=NOT  AllPortsSameDT=off  OutDataTypeStr=boolean
  Logical Operator2 : Logic  Operator=NOT  AllPortsSameDT=off  OutDataTypeStr=boolean
  Mux : Mux  Inputs=6
  Mux1 : Mux  Inputs=3
  PWM Generator (2-Level) : spsPWMGenerator2LevelLib/PWM Generator (2-Level)  ModulatorType=Three-phase bridge (6 pulses)  ModulatorMode=Unsynchronized  Fc=10000  Pc=90  nF=27  MinMax="[ -1  1 ]"  SamplingTechnique=Natural  ModulatingSignals=off  m=0.8  Freq=60  Phase=0  Ts=1e-6  ShowCarrierOutport=off
  PWM Reference Generator : mcbcontrolslib/PWM Reference Generator  inSignal=Valphabeta  modType=SVM: space vector modulation
      settings: LibrarySourceBlock=mcblib/Controls/Math Transforms/PWM Reference Generator
  Product : Product
  Product1 : Product
  Rate Limiter : RateLimiter  RisingSlewLimit=1000  SampleTimeMode=inherited
  Rate Transition : RateTransition  OutPortSampleTime=10e-5
  Scope : Scope  NumInputPorts=8
  Scope1 : Scope
  SpeedRef [RPM] : Step  Time=2  Before=500  After=1000  OutDataTypeStr=single  SampleTime=Ts
  Subsystem : Subsystem
  Terminator : Terminator
  Trigonometric Function : Trigonometry
  Trigonometric Function1 : Trigonometry  Operator=cos
  Unit Delay : UnitDelay  SampleTime=-1  HasFrameUpgradeWarning=on
  Out1 : Outport
  wires:
  SpeedRef [RPM]/1 -> Rate Limiter/1
  PWM Reference Generator/1 -> Mux1/1, Scope/6, Data Type Conversion1/1  "Va"
  PWM Reference Generator/2 -> Mux1/2, Scope/7, Data Type Conversion2/1  "Vb"
  Gain3/1 -> Product/1, Product1/1, Scope/3  "m"
  Gain2/1 -> Subsystem/1(fe)  "Ns_fe_we"
  Constant1/1 -> Add1/2
  Logical Operator2/1 -> Mux/6
  Data Type Conversion3/1 -> Mux/5, Logical Operator2/1
  Rate Transition/1 -> Gain3/1, Gain2/1
  Data Type Conversion2/1 -> Logical Operator1/1, Mux/3
  Product/1 -> Scope/5, PWM Reference Generator/2  "Vbeta"
  Trigonometric Function/1 -> Product/2
  Logical Operator/1 -> Mux/2
  Unit Delay/1 -> Subsystem/2(fb_teta)
  Mux/1 -> Terminator/1  "Dabc"
  Data Type Conversion1/1 -> Logical Operator/1, Mux/1
  Rate Limiter/1 -> Scope/1, Rate Transition/1  "N"
  Logical Operator1/1 -> Mux/4
  Add1/1 -> Trigonometric Function1/1, Trigonometric Function/1
  Product1/1 -> Scope/4, PWM Reference Generator/1  "Valpha"
  Trigonometric Function1/1 -> Product1/2
  PWM Reference Generator/3 -> Scope/8, Mux1/3, Data Type Conversion3/1  "Vc"
  PWM Generator (2-Level)/1 -> Scope1/1
  Constant/1 -> Out1/1
  Mux1/1 -> PWM Generator (2-Level)/1  "Dabc"
  Subsystem/1(tetaOL) -> Add1/1, Unit Delay/1, Scope/2  "Theta"

== system TestModel_V5_Timing_V2_2024a/Subsystem2 ==
  Pre_Mag_V1 : Subsystem  Commented=on
  Pre_Mag_V2 : Subsystem  Commented=on

== system TestModel_V5_Timing_V2_2024a/Subsystem3 ==
  Add4 : Sum  Inputs=+-
  Constant10 : Constant  Value=IM.Lm
  Constant9 : Constant  Value=IM.Lr
  Estimation : Subsystem
  RotorFluxEstimation : MATLAB Function  TreatAsAtomicUnit=on
  Scope : Scope  NumInputPorts=2
  Terminator{2..6} (5 alike) : Terminator
  wires:
  [IqSta] -> RotorFluxEstimation/2(IqSta)
  Constant9/1 -> RotorFluxEstimation/5(Lm)  "Lr"
  RotorFluxEstimation/2(psi_q_Rot) -> Terminator3/1  "psi_q_Rot"
  RotorFluxEstimation/3(psi_mag) -> Terminator4/1  "psi_mag"
  Add4/1 -> Terminator6/1  "theta_diff"
  Estimation/4(Speed_Est_MRAS) -> Scope/2  "Speed_Est_MRAS"
  Constant10/1 -> RotorFluxEstimation/6(Lr)  "Lm"
  [IqRot] -> RotorFluxEstimation/4(IqRot)
  RotorFluxEstimation/1(psi_d_Rot) -> Terminator2/1  "psi_d_Rot"
  Estimation/3(theta_est_MRAS) -> Scope/1  "theta_est_MRAS"
  [IdRot] -> RotorFluxEstimation/3(IdRot)
  [theta_e_mtr] -> Add4/1
  Estimation/2(Speed_Est_EBE) -> ?
  RotorFluxEstimation/4(Is) -> Terminator5/1  "Is"
  [theta_e] -> Add4/2
  ? -> RotorFluxEstimation/1(IdSta)
  Estimation/1(theta_est_EBE) -> ?

== system TestModel_V5_Timing_V2_2024a/Open_Loop/Subsystem ==
  note: Need to discuss about rate limitation block
  note: Ramp
  Constant4 : Constant  Commented=on  Value=50/15
  Constant6 : Constant  Commented=on  Value=10e-3
  MATLAB Function1 : MATLAB Function  Commented=on  TreatAsAtomicUnit=on
  MATLAB Function5 : MATLAB Function  Commented=on  TreatAsAtomicUnit=on
  Rate Transition : RateTransition  Commented=on  OutPortSampleTime=10e-3
  Speed_Rate : RateLimiter  Commented=on  RisingSlewLimit=par_Ctrl_SpdRt  FallingSlewLimit=-par_Ctrl_SpdRt  SampleTimeMode=inherited
  Unit Delay2 : UnitDelay  Commented=on  SampleTime=-1  HasFrameUpgradeWarning=on
  wires:
  Constant4/1 -> MATLAB Function1/2(ramp_rate)
  Constant6/1 -> MATLAB Function1/3(Ts)
  ? -> Rate Transition/1
  Unit Delay2/1 -> MATLAB Function5/2(data)
  MATLAB Function5/1(y) -> Unit Delay2/1  "F_e_Ramp"
  MATLAB Function1/1(y) -> ?
  Rate Transition/1 -> MATLAB Function1/1(speed_cmd)
  ? -> MATLAB Function5/1(u)
